simulink model "microgrid_top_fixed_final"  (R2025a)
settings: Solver=ode1  StartTime=0.0  StopTime=T_stop  FixedStep=Ts  RelTol=1e-3
InitFcn:
  | init_microgrid;
values from neighbouring files (symbols this model uses):
  C_dc = 25e-3    (= 0.025)    [init_microgrid.m]
  C_sc = 10    [init_microgrid.m]
  d = par.d    [init_microgrid.m]    (also in make_figures.m = diff([0; on; 0]))
  dt = t(2)-t(1)    [build_chb_inverter.m]    (also in init_microgrid.m = 0.25)
  Emax = 10    [init_microgrid.m]
  eta_inv = 0.96    [init_microgrid.m]
  Ki_ib = Kp_ib*2*pi*fc_i/10    (= 11.8435252813)    [init_microgrid.m]
  Ki_isc = Kp_isc*2*pi*fc_i/10    (= 14.0148382495)    [init_microgrid.m]
  Ki_v = Kp_v*2*pi*fv/10    (= 63.165468167)    [init_microgrid.m]
  Kp_ib = 2*pi*fc_i*L_bat/V_dc_ref    (= 0.00942477796077)    [init_microgrid.m]
  Kp_isc = 2*pi*fc_i*L_sc/V_dc_ref    (= 0.0111526539202)    [init_microgrid.m]
  Kp_v = 2*pi*fv*C_dc*V_dc_ref/V_sc_nom    (= 5.02654824574)    [init_microgrid.m]
  LOAD_SIGN = +1    (= 1)    [init_microgrid.m]
  Pbmax = par.Pb_max    [init_microgrid.m]
  Pmax = max(Ph,[],2)'    [init_microgrid.m]
  prof = Ph'    [init_microgrid.m]    (also in make_figures.m = evalin('base','prof'); end)
  Pscale = 1    [init_microgrid.m]
  Q_sim_Ah = Q_real_Ah*k_scale    (= 0.0180555555556)    [init_microgrid.m]
  R_bat = 0.05    [init_microgrid.m]
  sig = [0.03 0.10 0.15]    [init_microgrid.m]    (also in ppt_plots_pv.m = {Vpv, Ipv, Ppv, Dty, Vbus})
  SoC0 = par.SoC_0    [init_microgrid.m]
  SoC_min = par.SoC_min    [init_microgrid.m]
  T_amb_day = T_amb_cloudy_day; else, G_day = G_clear_day; end    [init_microgrid.m]    (also in run_test1_pv.m = S.T_amb; end\n']))
  t_day = S.t    [init_microgrid.m]
  t_hour = 0.12    [init_microgrid.m]    (also in plot_test4.m = evalin('base','t_hour'); ppt_plots_pv.m = 0.05)
  tau_lpf = 2e-3    (= 0.002)    [init_microgrid.m]
  Tc = 2    [init_microgrid.m]    (also in ppt_plots_pv.m = squeeze(wx.getElement(2).Values.Data))
  th1 = par.th1    [init_microgrid.m]    (also in make_figures.m = 0.05)
  th1_act = th1    [init_microgrid.m]
  th2 = par.th2    [init_microgrid.m]
  th2_act = th2    [init_microgrid.m]
  Ts = Ts_pwr    (= 1e-06)    [init_microgrid.m]
  Ts_ems = t_hour/60    (= 0.002)    [init_microgrid.m]
  Ts_fc = dt*t_hour    (= 0.03)    [init_microgrid.m]
  V_bat_nom = 240    [init_microgrid.m]
  V_dc_ref = 400    [init_microgrid.m]
  V_sc_nom = 250    [init_microgrid.m]
undefined symbols (not defined in the file or in its folder): DiscIntNeverNeededParam, G_day, Ion, Lithium
libraries: spsSeriesRLCBranchLib x9, slpidlib x5, spsVoltageMeasurementLib x5, spsIdealSwitchLib x5, spsIGBTDiodeLib x4, spsCurrentMeasurementLib x3, simulink x3, spsParallelRLCLoadLib x3, spsPWMGeneratorDCDCLib x2, spsDiodeLib x2, spsPVArrayLib x2, spsBatteryLib x1
(part 1 of 2)
settings Model: Creator=mdnih  LastModifiedBy=msssr
settings SolverCC: AutoInsertRateTranBlk=on
settings DebuggingCC: UnconnectedInputMsg=warning

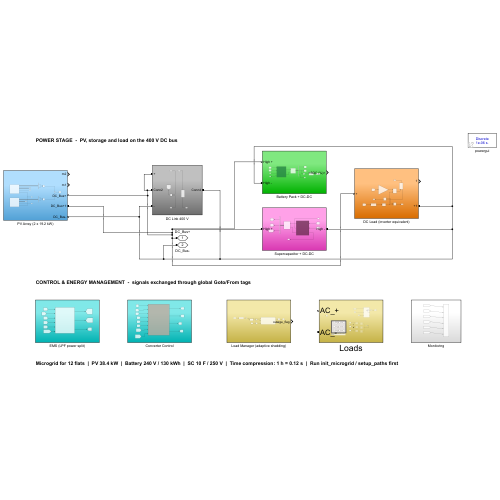
[thumbnail: Simulink's stored preview of the top-level diagram]
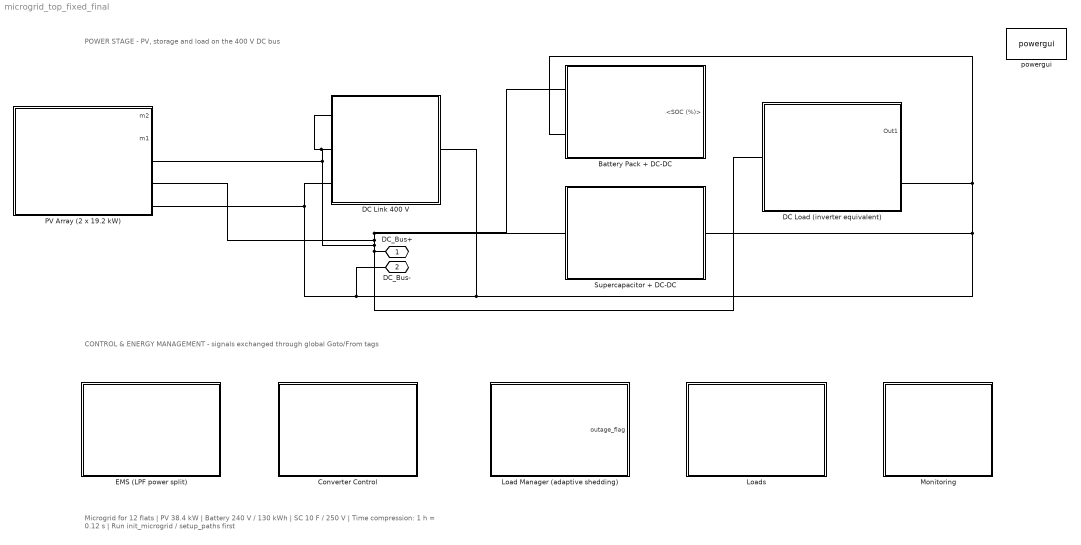
== system microgrid_top_fixed_final ==
  note: POWER STAGE - PV, storage and load on the 400 V DC bus
  note: CONTROL & ENERGY MANAGEMENT - signals exchanged through global Goto/From tags
  note: Microgrid for 12 flats | PV 38.4 kW | Battery 240 V / 130 kWh | SC 10 F / 250 V | Time compression: 1 h = 0.12 s | Run init_microgrid / setup_paths first
  Battery Pack + DC-DC : Subsystem
  Converter Control : Subsystem
  DC Link 400 V : Subsystem
  DC Load (inverter equivalent) : Subsystem
  EMS (LPF power split) : Subsystem
  Load Manager (adaptive shedding) : Subsystem
  Loads : Subsystem
  Monitoring : Subsystem
  PV Array (2 x 19.2 kW) : Subsystem
  Supercapacitor + DC-DC : Subsystem
  powergui : sps_lib/powergui  Priority=1  SimulationMode=Discrete  SampleTime=Ts  frequency=60  Iterations=50  frequencyindice=0  Pbase=100e6  ErrMax=1e-4  UnitsV=kV  UnitsW=MW  buscounter=0  FunctionMessages=off  echomessages=off  EnableUseOfTLC=off  CurrentSourceSwitches=off  DisableSnubberDevices=off  DisableRonSwitches=off  DisableVfSwitches=off  DisplayEquations=off  AutomaticDiscreteSolvers=off  SolverType=Tustin/Backward Euler (TBE)  Interpol=off  ExternalGateDelay=off  methode=off  Ts=100  x0status=blocks  SPID=on  SwTol=0  HookPort=off  NonlinearTolerance=1e-4  nMaxIteration=100  ContinueOnMaxIteration=off  RestoreLinks=warning  ResistiveCurrentMeasurement=off  Frange=[0:2:500]  Ylog=off  Xlog=on  ShowGrid=off  save=off  variable=ZData  structure=0  ZoomFFT=off  StartTime=0.0  cycles=1  DisplayStyle=1  fundamental=60  FreqAxis=off  MaxFrequency=1000  frequencyindicesteady=1  RmsSteady=1  display=off
  DC_Bus+ : PMIOPort  Side=Right
  DC_Bus- : PMIOPort  Port=2  Side=Left
  connections:
  DC Link 400 V/LConn2 -- DC Link 400 V/LConn1 -- PV Array (2 x 19.2 kW)/RConn2 -- Battery Pack + DC-DC/LConn1 -- Supercapacitor + DC-DC/LConn1 -- DC Load (inverter equivalent)/LConn1 -- DC_Bus+/RConn1 -- PV Array (2 x 19.2 kW)/RConn1
  PV Array (2 x 19.2 kW)/RConn3 -- DC Load (inverter equivalent)/RConn1 -- Battery Pack + DC-DC/LConn2 -- Supercapacitor + DC-DC/RConn1 -- DC Link 400 V/RConn1 -- DC_Bus-/RConn1 -- DC Link 400 V/LConn3

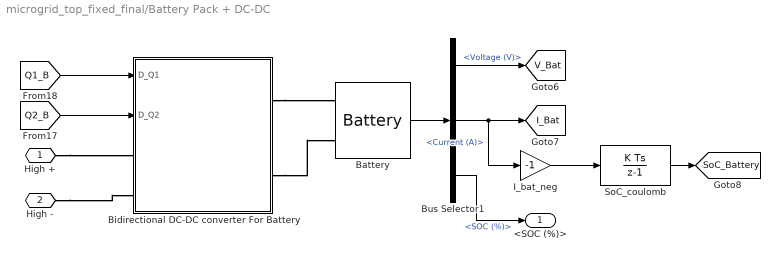
== system microgrid_top_fixed_final/Battery Pack + DC-DC ==
  Battery : spsBatteryLib/Battery  BatType=Lithium-Ion  NomV=V_bat_nom  NomQ=Q_real_Ah  SOC=SoC0*100  Batt_Tr=1e-3  PresetModel=off  MaxQ=Q_real_Ah  MinV=180  FullV=279.3569  Dis_rate=235.5072  R=R_bat  Normal_OP=489.8551  expZone="[259.2926      26.61232]"
      settings: LibrarySourceBlock=electricdrivelib/Extra Sources/Battery
  Bidirectional DC-DC converter For Battery : Subsystem
  Bus Selector1 : BusSelector  OutputSignals=Voltage (V),Current (A),SOC (%)
  I_bat_neg : Gain  Gain=-1
  SoC_coulomb : DiscreteIntegrator  gainval=100/(3600*Q_sim_Ah)  InitialCondition=SoC0*100  SampleTime=Ts  LimitOutput=on  UpperSaturationLimit=100  LowerSaturationLimit=0  ICPrevOutput=DiscIntNeverNeededParam  ICPrevScaledInput=DiscIntNeverNeededParam
  High + : PMIOPort  Side=Left
  High - : PMIOPort  Port=2  Side=Left
  <SOC (%)> : Outport
  tag scope: I_Bat=global, SoC_Battery=global, V_Bat=global
  wires:
  [Q2_B] -> Bidirectional DC-DC converter For Battery/2(D_Q2)
  [Q1_B] -> Bidirectional DC-DC converter For Battery/1(D_Q1)
  Bus Selector1/1 -> [V_Bat]  "<Voltage (V)>"
  I_bat_neg/1 -> SoC_coulomb/1
  Battery/1 -> Bus Selector1/1
  Bus Selector1/2 -> I_bat_neg/1, [I_Bat]  "<Current (A)>"
  Bus Selector1/3 -> <SOC (%)>/1  "<SOC (%)>"
  SoC_coulomb/1 -> [SoC_Battery]
  connections:
  High +/RConn1 -- Bidirectional DC-DC converter For Battery/LConn1
  Bidirectional DC-DC converter For Battery/RConn1 -- Battery/LConn1
  High -/RConn1 -- Bidirectional DC-DC converter For Battery/LConn2
  Bidirectional DC-DC converter For Battery/RConn2 -- Battery/LConn2

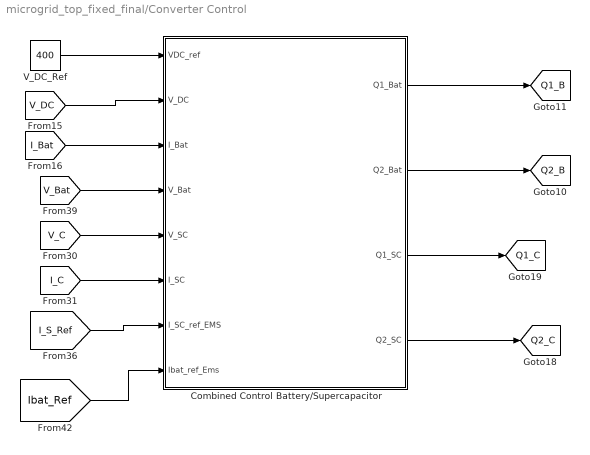
== system microgrid_top_fixed_final/Converter Control ==
  Combined Control Battery/Supercapacitor : Subsystem
  V_DC_Ref : Constant  Value=400
  tag scope: Q1_B=global, Q1_C=global, Q2_B=global, Q2_C=global
  wires:
  [I_C] -> Combined Control Battery/Supercapacitor/6(I_SC)
  [V_DC] -> Combined Control Battery/Supercapacitor/2(V_DC)
  Combined Control Battery/Supercapacitor/4(Q2_SC) -> [Q2_C]
  Combined Control Battery/Supercapacitor/1(Q1_Bat) -> [Q1_B]
  Combined Control Battery/Supercapacitor/3(Q1_SC) -> [Q1_C]
  [I_S_Ref] -> Combined Control Battery/Supercapacitor/7(I_SC_ref_EMS)
  [Ibat_Ref] -> Combined Control Battery/Supercapacitor/8(Ibat_ref_Ems)
  Combined Control Battery/Supercapacitor/2(Q2_Bat) -> [Q2_B]
  V_DC_Ref/1 -> Combined Control Battery/Supercapacitor/1(VDC_ref)
  [I_Bat] -> Combined Control Battery/Supercapacitor/3(I_Bat)
  [V_C] -> Combined Control Battery/Supercapacitor/5("V_SC ")
  [V_Bat] -> Combined Control Battery/Supercapacitor/4(V_Bat)

== system microgrid_top_fixed_final/DC Link 400 V ==
  C_DC_Link : spsSeriesRLCBranchLib/Series RLC Branch  LConnTagsString=__new0  RConnTagsString=__new0  BranchType=C  Resistance=1  Inductance=1e-3  SetiL0=off  InitialCurrent=0  Capacitance=C_dc  Setx0=off  InitialVoltage=0  Measurements=None
  Voltage Measurement : spsVoltageMeasurementLib/Voltage Measurement  PhasorSimulation=off  OutputType=Complex  PSBequivalent=0
  + : PMIOPort  Side=Left
  Conn2 : PMIOPort  Port=2  Side=Left
  - : PMIOPort  Port=3  Side=Left
  Conn4 : PMIOPort  Port=4  Side=Right
  tag scope: V_DC=global
  wires:
  Voltage Measurement/1 -> [V_DC]
  connections:
  C_DC_Link/RConn1 -- Conn4/RConn1
  C_DC_Link/LConn1 -- Conn2/RConn1
  Voltage Measurement/LConn1 -- +/RConn1
  Voltage Measurement/LConn2 -- -/RConn1

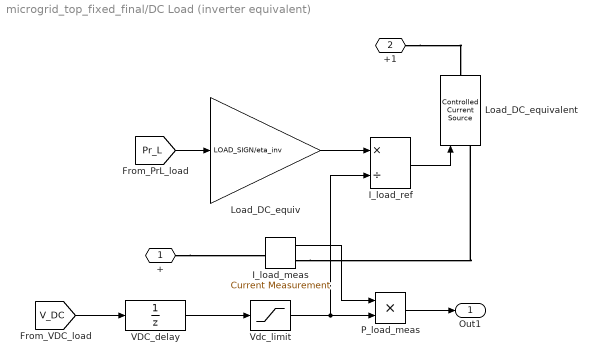
== system microgrid_top_fixed_final/DC Load (inverter equivalent) ==
  I_load_meas : spsCurrentMeasurementLib/Current Measurement  PhasorSimulation=off  OutputType=Complex  PSBequivalent=0
  I_load_ref : Product  Inputs=*/
  Load_DC_equiv : Gain  Gain=LOAD_SIGN/eta_inv
  Load_DC_equivalent : spsControlledCurrentSourceLib/Controlled Current Source  Initialize=on  Source_Type=AC  Amplitude=0  Phase=0  Frequency=0  Measurements=None
  P_load_meas : Product
  VDC_delay : UnitDelay  InitialCondition=V_dc_ref  SampleTime=Ts  HasFrameUpgradeWarning=on
  Vdc_limit : Saturate  UpperLimit=450  LowerLimit=300
  + : PMIOPort  Side=Left
  +1 : PMIOPort  Port=2  Side=Right
  Out1 : Outport
  wires:
  [Pr_L] -> Load_DC_equiv/1
  [V_DC] -> VDC_delay/1
  VDC_delay/1 -> Vdc_limit/1
  Load_DC_equiv/1 -> I_load_ref/1
  I_load_meas/1 -> P_load_meas/1
  Vdc_limit/1 -> I_load_ref/2, P_load_meas/2
  I_load_ref/1 -> Load_DC_equivalent/1
  P_load_meas/1 -> Out1/1
  connections:
  I_load_meas/RConn1 -- Load_DC_equivalent/LConn1
  +/RConn1 -- I_load_meas/LConn1
  +1/RConn1 -- Load_DC_equivalent/RConn1

== system microgrid_top_fixed_final/EMS (LPF power split) ==
  BESS : Subsystem
  tag scope: I_S_Ref=global, Ibat_Ref=global, P_DEF=global
  wires:
  BESS/1(I_BAT_REF) -> [Ibat_Ref]
  [Pr_L] -> BESS/1(P_L)
  [V_Bat] -> BESS/3(V_BAT)
  [P_PV] -> BESS/2(p_pv)
  [I_C] -> BESS/5(I_C)
  [SoC_Battery] -> BESS/6(SOC_Bat)
  [V_C] -> BESS/4(V_C)
  BESS/2(I_S_REF) -> [I_S_Ref]
  BESS/3(P_DEF) -> [P_DEF]

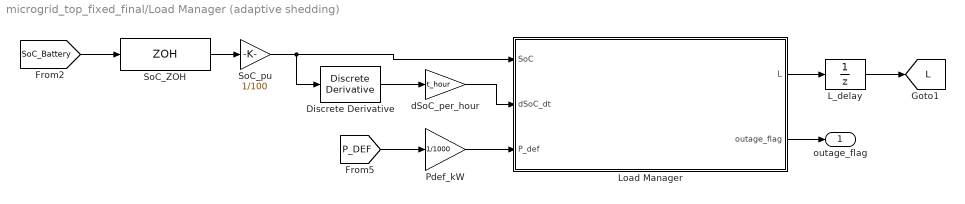
== system microgrid_top_fixed_final/Load Manager (adaptive shedding) ==
  Discrete Derivative : simulink/Discrete/Discrete Derivative  gainval=1.0  ICPrevScaledInput=0.0  OutMin=[]  OutMax=[]  OutDataType=fixdt(1, 16)  OutScaling=2^-10  DoSatur=off
  L_delay : UnitDelay  SampleTime=Ts_ems  HasFrameUpgradeWarning=on
  Load Manager : Stateflow chart  TreatAsAtomicUnit=on
  Pdef_kW : Gain  Gain=1/1000
  SoC_ZOH : ZeroOrderHold  SampleTime=Ts_ems
  SoC_pu : Gain  Gain=1/100
  dSoC_per_hour : Gain  Gain=t_hour
  outage_flag : Outport
  tag scope: L=global
  wires:
  Discrete Derivative/1 -> dSoC_per_hour/1
  [SoC_Battery] -> SoC_ZOH/1
  SoC_ZOH/1 -> SoC_pu/1
  Pdef_kW/1 -> Load Manager/3(P_def)
  SoC_pu/1 -> Load Manager/1(SoC), Discrete Derivative/1
  [P_DEF] -> Pdef_kW/1
  dSoC_per_hour/1 -> Load Manager/2(dSoC_dt)
  Load Manager/1(L) -> L_delay/1
  Load Manager/2(outage_flag) -> outage_flag/1
  L_delay/1 -> [L]

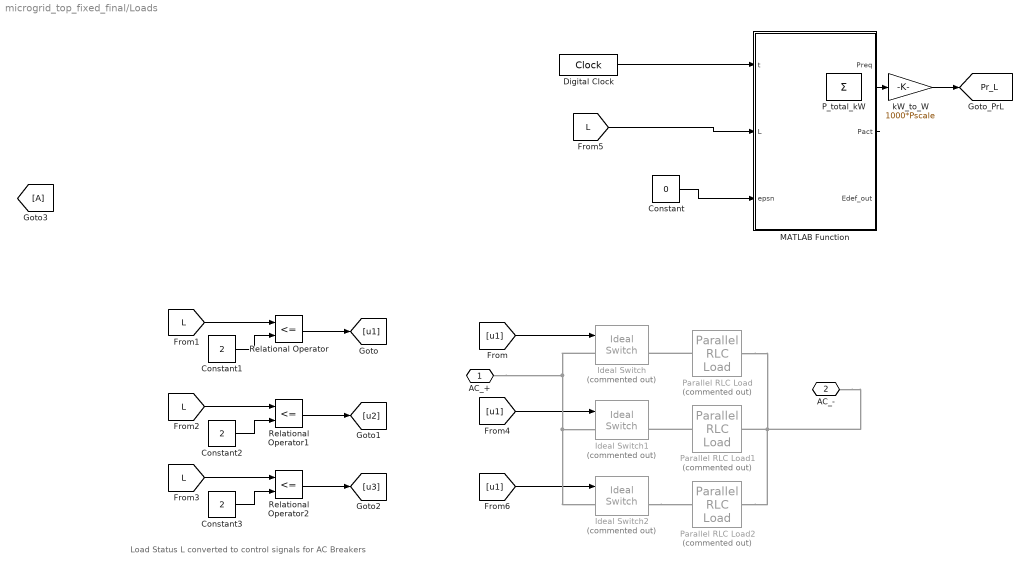
== system microgrid_top_fixed_final/Loads ==
  note: Load Status L converted to control signals
      | for AC Breakers
  Constant : Constant  Value=0
  Constant1 : Constant  Value=2
  Constant2 : Constant  Value=2
  Constant3 : Constant  Value=2
  Digital Clock : DigitalClock  SampleTime=Ts_fc
  Goto3 : Goto
  Ideal Switch : spsIdealSwitchLib/Ideal Switch  Commented=on  Ron=0.001  Lon=0  IC=0  Rs=1e5  Cs=inf  Measurements=on
  Ideal Switch1 : spsIdealSwitchLib/Ideal Switch  Commented=on  Ron=0.001  Lon=0  IC=0  Rs=1e5  Cs=inf  Measurements=on
  Ideal Switch2 : spsIdealSwitchLib/Ideal Switch  Commented=on  Ron=0.001  Lon=0  IC=0  Rs=1e5  Cs=inf  Measurements=on
  MATLAB Function : MATLAB Function  TreatAsAtomicUnit=on
  P_total_kW : Sum  Inputs=+
  Parallel RLC Load : spsParallelRLCLoadLib/Parallel RLC Load  Commented=on  LConnTagsString=a  RConnTagsString=__new0  NominalVoltage=1000  NominalFrequency=60  ActivePower=10e3  InductivePower=100  CapacitivePower=100  Setx0=off  InitialVoltage=0  SetiL0=off  InitialCurrent=0  Measurements=None  LoadType=constant Z
      settings: AttributesFormatString=\n  LibrarySourceBlock=sps_lib/Passives/Parallel RLC Load
  Parallel RLC Load1 : spsParallelRLCLoadLib/Parallel RLC Load  Commented=on  LConnTagsString=a  RConnTagsString=__new0  NominalVoltage=1000  NominalFrequency=60  ActivePower=10e3  InductivePower=100  CapacitivePower=100  Setx0=off  InitialVoltage=0  SetiL0=off  InitialCurrent=0  Measurements=None  LoadType=constant Z
      settings: AttributesFormatString=\n  LibrarySourceBlock=sps_lib/Passives/Parallel RLC Load
  Parallel RLC Load2 : spsParallelRLCLoadLib/Parallel RLC Load  Commented=on  LConnTagsString=a  RConnTagsString=__new0  NominalVoltage=1000  NominalFrequency=60  ActivePower=10e3  InductivePower=100  CapacitivePower=100  Setx0=off  InitialVoltage=0  SetiL0=off  InitialCurrent=0  Measurements=None  LoadType=constant Z
      settings: AttributesFormatString=\n  LibrarySourceBlock=sps_lib/Passives/Parallel RLC Load
  Relational Operator : RelationalOperator  Operator=<=  OutDataTypeStr=boolean  RndMeth=Simplest  InputSameDT=off
  Relational Operator1 : RelationalOperator  Operator=<=  OutDataTypeStr=boolean  RndMeth=Simplest  InputSameDT=off
  Relational Operator2 : RelationalOperator  Operator=<=  OutDataTypeStr=boolean  RndMeth=Simplest  InputSameDT=off
  kW_to_W : Gain  Gain=1000*Pscale
  AC_+ : PMIOPort  Side=Left
  AC_- : PMIOPort  Port=2  Side=Left
  tag scope: Pr_L=global
  wires:
  Digital Clock/1 -> MATLAB Function/1(t)
  [L] -> MATLAB Function/2(L)
  Constant/1 -> MATLAB Function/3(epsn)
  [L] -> Relational Operator/1
  Constant1/1 -> Relational Operator/2
  Constant2/1 -> Relational Operator1/2
  [L] -> Relational Operator1/1
  [L] -> Relational Operator2/1
  Constant3/1 -> Relational Operator2/2
  Relational Operator/1 -> [u1]
  Relational Operator2/1 -> [u3]
  Relational Operator1/1 -> [u2]
  [u1] -> Ideal Switch/1
  [u1] -> Ideal Switch1/1
  [u1] -> Ideal Switch2/1
  MATLAB Function/2(Pact) -> P_total_kW/1
  P_total_kW/1 -> kW_to_W/1
  kW_to_W/1 -> [Pr_L]
  connections:
  Ideal Switch/LConn1 -- Ideal Switch2/LConn1 -- Ideal Switch1/LConn1 -- AC_+/RConn1
  Parallel RLC Load/LConn1 -- Ideal Switch/RConn1
  Parallel RLC Load1/LConn1 -- Ideal Switch1/RConn1
  Ideal Switch2/RConn1 -- Parallel RLC Load2/LConn1
  Parallel RLC Load/RConn1 -- AC_-/RConn1 -- Parallel RLC Load1/RConn1 -- Parallel RLC Load2/RConn1

== system microgrid_top_fixed_final/Monitoring ==
  System Scope : Scope  NumInputPorts=6
      settings: ActiveDisplayYMinimum=89.7017199795797  ActiveDisplayYMaximum=442.12734403903488
  wires:
  [V_DC] -> System Scope/1
  [V_Bat] -> System Scope/2
  [SoC_Battery] -> System Scope/3
  [P_PV] -> System Scope/4
  [Pr_L] -> System Scope/5
  [L] -> System Scope/6

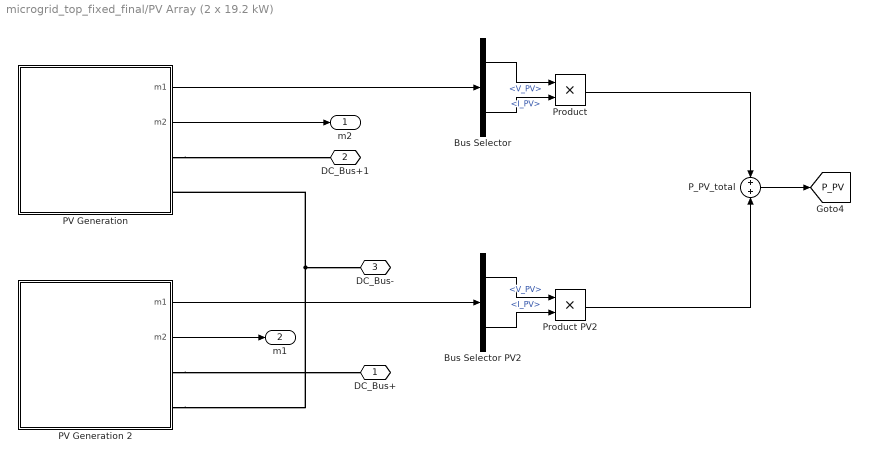
== system microgrid_top_fixed_final/PV Array (2 x 19.2 kW) ==
  Bus Selector : BusSelector  OutputSignals=V_PV,I_PV
  Bus Selector PV2 : BusSelector  OutputSignals=V_PV,I_PV
  PV Generation : Subsystem
  PV Generation 2 : Subsystem
  P_PV_total : Sum
  Product : Product
  Product PV2 : Product
  DC_Bus+ : PMIOPort  Side=Right
  DC_Bus+1 : PMIOPort  Port=2  Side=Right
  DC_Bus- : PMIOPort  Port=3  Side=Right
  m2 : Outport
  m1 : Outport  Port=2
  tag scope: P_PV=global
  wires:
  P_PV_total/1 -> [P_PV]
  Bus Selector PV2/2 -> Product PV2/2  "<I_PV>"
  PV Generation 2/1(m1) -> Bus Selector PV2/1
  PV Generation 2/2(m2) -> m1/1
  PV Generation/2(m2) -> m2/1
  PV Generation/1(m1) -> Bus Selector/1
  Bus Selector PV2/1 -> Product PV2/1  "<V_PV>"
  Product PV2/1 -> P_PV_total/2
  Bus Selector/1 -> Product/1  "<V_PV>"
  Bus Selector/2 -> Product/2  "<I_PV>"
  Product/1 -> P_PV_total/1
  connections:
  PV Generation 2/RConn1 -- DC_Bus+/RConn1
  PV Generation 2/RConn2 -- PV Generation/RConn2 -- DC_Bus-/RConn1
  PV Generation/RConn1 -- DC_Bus+1/RConn1

== system microgrid_top_fixed_final/Supercapacitor + DC-DC ==
  Bidirectional DC-DC converter For Supercapacitor : Subsystem
  Bus Selector2 : BusSelector  OutputSignals=Voltage V,Current I,SOC %
  Supercapacitor : spsSupercapacitorLib/Supercapacitor  C=C_sc  Rdc=0.003  Voltage=V_sc_nom  Ns=1  Np=1  Vinit=V_sc_init  Temp=25  Nc=1  r=1e-9  epsilon=6.0208e-10  Ioc=10  Vself="[48  47.8  47.06  44.65]"
      settings: LibrarySourceBlock=electricdrivelib/Extra Sources/Supercapacitor
  High + : PMIOPort  Side=Left
  High - : PMIOPort  Port=2  Side=Right
  tag scope: I_C=global, SoC_Cap=global, V_C=global
  wires:
  Bus Selector2/3 -> [SoC_Cap]  "<SOC %>"
  Bus Selector2/2 -> [I_C]  "<Current I>"
  Supercapacitor/1 -> Bus Selector2/1
  Bus Selector2/1 -> [V_C]  "<Voltage V>"
  [Q1_C] -> Bidirectional DC-DC converter For Supercapacitor/1(D_Q1)
  [Q2_C] -> Bidirectional DC-DC converter For Supercapacitor/2(D_Q2)
  connections:
  High -/RConn1 -- Bidirectional DC-DC converter For Supercapacitor/RConn2
  High +/RConn1 -- Bidirectional DC-DC converter For Supercapacitor/LConn1
  Supercapacitor/LConn1 -- Bidirectional DC-DC converter For Supercapacitor/RConn1
  Supercapacitor/LConn2 -- Bidirectional DC-DC converter For Supercapacitor/RConn3

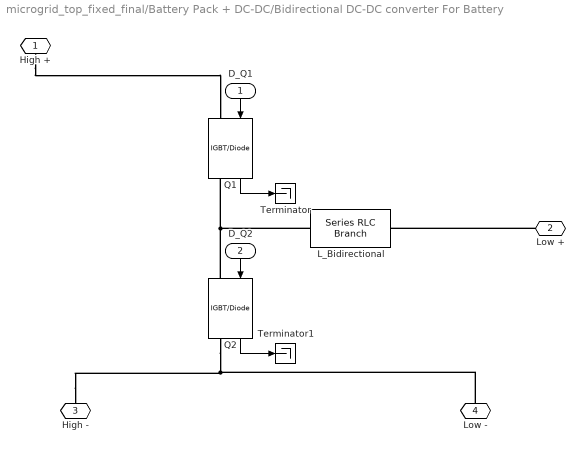
== system microgrid_top_fixed_final/Battery Pack + DC-DC/Bidirectional DC-DC converter For Battery ==
  D_Q1 : Inport
  D_Q2 : Inport  Port=2
  L_Bidirectional : spsSeriesRLCBranchLib/Series RLC Branch  LConnTagsString=__new0  RConnTagsString=__new0  BranchType=RL  Resistance=0.05  Inductance=0.3e-3  SetiL0=off  InitialCurrent=0  Capacitance=1e-6  Setx0=off  InitialVoltage=0  Measurements=None
  Q1 : spsIGBTDiodeLib/IGBT//Diode  Ron=1e-3  Rs=1e5  Cs=inf  Measurements=on
  Q2 : spsIGBTDiodeLib/IGBT//Diode  Ron=1e-3  Rs=1e5  Cs=inf  Measurements=on
  Terminator : Terminator
  Terminator1 : Terminator
  High + : PMIOPort  Side=Left
  Low + : PMIOPort  Port=2  Side=Right
  High - : PMIOPort  Port=3  Side=Left
  Low - : PMIOPort  Port=4  Side=Right
  wires:
  D_Q2/1 -> Q2/1
  D_Q1/1 -> Q1/1
  Q1/1 -> Terminator/1
  Q2/1 -> Terminator1/1
  connections:
  High -/RConn1 -- Low -/RConn1 -- Q2/RConn1
  High +/RConn1 -- Q1/LConn1
  Low +/RConn1 -- L_Bidirectional/RConn1
  Q2/LConn1 -- L_Bidirectional/LConn1 -- Q1/RConn1

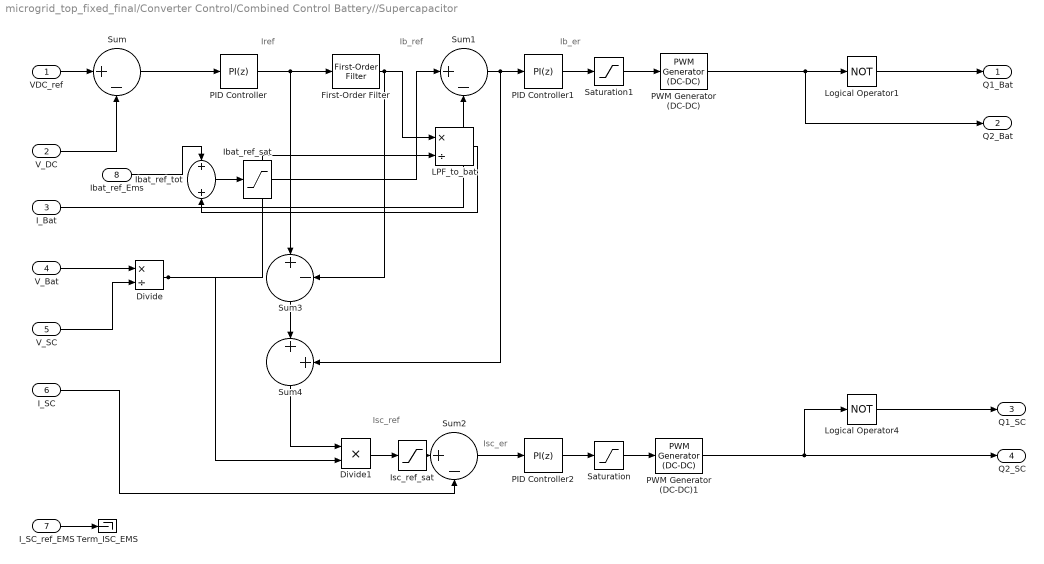
== system microgrid_top_fixed_final/Converter Control/Combined Control Battery//Supercapacitor ==
  note: Isc_er
  note: Isc_ref
  note: Ib_er
  note: Ib_ref
  note: Iref
  VDC_ref : Inport
  V_DC : Inport  Port=2
  I_Bat : Inport  Port=3
  V_Bat : Inport  Port=4
  "V_SC " : Inport  Port=5
  I_SC : Inport  Port=6
  I_SC_ref_EMS : Inport  Port=7
  Ibat_ref_Ems : Inport  Port=8
  Divide : Product  Inputs=*/
  Divide1 : Product  Inputs=**
  First-Order Filter : spsFirstOrderFilterLib/First-Order Filter  FilterType=Lowpass  Tc=0.015  Ts=Ts  Initialize=off  Vac_Init=[0, 0, 60]  Vdc_Init=0  PlotResponse=off  FreqRange="[0,  200,  1]"
  Ibat_ref_sat : Saturate  UpperLimit=1.5*Pbmax*1e3/V_bat_nom  LowerLimit=-(1.5*Pbmax*1e3/V_bat_nom)
  Ibat_ref_tot : Sum
  Isc_ref_sat : Saturate  UpperLimit=200  LowerLimit=-(200)
  LPF_to_bat : Product  Inputs=*/
  Logical Operator1 : Logic  Operator=NOT  AllPortsSameDT=off  OutDataTypeStr=boolean
  Logical Operator4 : Logic  Operator=NOT  AllPortsSameDT=off  OutDataTypeStr=boolean
  PID Controller : slpidlib/PID Controller  Controller=PI  Form=Parallel  TimeDomain=Discrete-time  UseExternalTs=off  SampleTime=Ts  IntegratorMethod=Backward Euler  FilterMethod=Backward Euler  ControllerParametersSource=internal  P=Kp_v  I=Ki_v  UseKiTs=off  D=0  UseExternalDerivativeSource=off  N=100  UseFilter=on  TunerSelectOption=Transfer Function Based (PID Tuner App)  InitialConditionSource=internal  InitialConditionForIntegrator=0  InitialConditionForFilter=0  DifferentiatorICPrevScaledInput=0  ExternalReset=none  TrackingMode=off  Kt=1  LimitOutput=on  SatLimitsSource=internal  UpperSaturationLimit=1.5*Pbmax*1e3/V_bat_nom + 200  LowerSaturationLimit=-(1.5*Pbmax*1e3/V_bat_nom + 200)  LinearizeAsGain=on  AntiWindupMode=clamping  Kb=1  LimitIntegrator=off  UpperIntegratorSaturationLimit=inf  LowerIntegratorSaturationLimit=-inf  POutMin=[]  POutMax=[]  IOutMin=[]  IOutMax=[]  DOutMin=[]  DOutMax=[]  NOutMin=[]  NOutMax=[]  SumOutMin=[]  SumOutMax=[]  SaturationOutMin=[]  SaturationOutMax=[]  PParamMin=[]  PParamMax=[]  IParamMin=[]  IParamMax=[]  DParamMin=[]  DParamMax=[]  NParamMin=[]  NParamMax=[]  KbParamMin=[]  KbParamMax=[]  KtParamMin=[]  KtParamMax=[]  KbOutMin=[]  KbOutMax=[]  KtOutMin=[]  KtOutMax=[]  IntegratorOutMin=[]  IntegratorOutMax=[]  FilterOutMin=[]  FilterOutMax=[]  SumI1OutMin=[]  SumI1OutMax=[]  SumI2OutMin=[]  SumI2OutMax=[]  SumI3OutMin=[]  SumI3OutMax=[]  SumI4OutMin=[]  SumI4OutMax=[]  SumDOutMin=[]  SumDOutMax=[]  DifferentiatorOutMin=[]  DifferentiatorOutMax=[]  FilterDiffOutCoefMin=[]  FilterDiffOutCoefMax=[]  ReciprocalOutMin=[]  ReciprocalOutMax=[]  SumDenOutMin=[]  SumDenOutMax=[]  SumNumOutMin=[]  SumNumOutMax=[]  DivideOutMin=[]  DivideOutMax=[]  UdiffTsProdOutMin=[]  UdiffTsProdOutMax=[]  NTsProdOutMin=[]  NTsProdOutMax=[]  UintegralTsProdOutMin=[]  UintegralTsProdOutMax=[]  UngainTsProdOutMin=[]  UngainTsProdOutMax=[]  ClampingZeroOutDataTypeStr=Inherit: Inherit via back propagation  ClampingZeroOutMin=[]  ClampingZeroOutMax=[]  FilterDenConstantOutDataTypeStr=Inherit: Inherit via back propagation  FilterDenConstantOutMin=[]  FilterDenConstantOutMax=[]  PCopyOutDataTypeStr=Inherit: Inherit via back propagation  PCopyOutMin=[]  PCopyOutMax=[]  NCopyOutDataTypeStr=Inherit: Inherit via back propagation  NCopyOutMin=[]  NCopyOutMax=[]  IntegratorContinuousStateAttributes=''  IntegratorStateMustResolveToSignalObject=off  IntegratorRTWStateStorageClass=Auto  FilterContinuousStateAttributes=''  FilterStateMustResolveToSignalObject=off  FilterRTWStateStorageClass=Auto  ParallelPVariant=InternalParameters  IdealPVariant=Disabled  IVariant=InternalParameters  DVariant=Disabled  IntegratorVariant=Discrete  SatVariant=Enabled  AWVariant=DiscClampingParallel  PCopyVariant=Disabled  TRVariant=Disabled  FdbkBlocksVariant=Feedback  IdealPFdbkVariant=Passthrough  SatFdbkVariant=Passthrough  DerivativeFilterVariant=Disabled  NVariant=Disabled  NCopyVariant=Disabled_SignalSpec  FilterICVariant=Disabled  IntegratorICVariant=InternalICs  ExternalResetVariant=Disabled  TRSumVariant=Passthrough  SumFdbkVariant=Enabled  SumVariant=Sum_PI  TsampFilterVariant=InternalTs  TsampNgainVariant=Passthrough  TsampIntegralVariant=Disabled_SignalSpec  ExternalSaturationOutDataTypeStr=Inherit: Same as second input  DerivativeSourceVariant=Disabled  PreIntVariant=InternalPreInt
  PID Controller1 : slpidlib/PID Controller  Controller=PI  Form=Parallel  TimeDomain=Discrete-time  UseExternalTs=off  SampleTime=Ts  IntegratorMethod=Backward Euler  FilterMethod=Backward Euler  ControllerParametersSource=internal  P=Kp_ib  I=Ki_ib  UseKiTs=off  D=0  UseExternalDerivativeSource=off  N=100  UseFilter=on  TunerSelectOption=Transfer Function Based (PID Tuner App)  InitialConditionSource=internal  InitialConditionForIntegrator=0  InitialConditionForFilter=0  DifferentiatorICPrevScaledInput=0  ExternalReset=none  TrackingMode=off  Kt=1  LimitOutput=on  SatLimitsSource=internal  UpperSaturationLimit=0.9  LowerSaturationLimit=0  LinearizeAsGain=on  AntiWindupMode=clamping  Kb=1  LimitIntegrator=off  UpperIntegratorSaturationLimit=inf  LowerIntegratorSaturationLimit=-inf  POutMin=[]  POutMax=[]  IOutMin=[]  IOutMax=[]  DOutMin=[]  DOutMax=[]  NOutMin=[]  NOutMax=[]  SumOutMin=[]  SumOutMax=[]  SaturationOutMin=[]  SaturationOutMax=[]  PParamMin=[]  PParamMax=[]  IParamMin=[]  IParamMax=[]  DParamMin=[]  DParamMax=[]  NParamMin=[]  NParamMax=[]  KbParamMin=[]  KbParamMax=[]  KtParamMin=[]  KtParamMax=[]  KbOutMin=[]  KbOutMax=[]  KtOutMin=[]  KtOutMax=[]  IntegratorOutMin=[]  IntegratorOutMax=[]  FilterOutMin=[]  FilterOutMax=[]  SumI1OutMin=[]  SumI1OutMax=[]  SumI2OutMin=[]  SumI2OutMax=[]  SumI3OutMin=[]  SumI3OutMax=[]  SumI4OutMin=[]  SumI4OutMax=[]  SumDOutMin=[]  SumDOutMax=[]  DifferentiatorOutMin=[]  DifferentiatorOutMax=[]  FilterDiffOutCoefMin=[]  FilterDiffOutCoefMax=[]  ReciprocalOutMin=[]  ReciprocalOutMax=[]  SumDenOutMin=[]  SumDenOutMax=[]  SumNumOutMin=[]  SumNumOutMax=[]  DivideOutMin=[]  DivideOutMax=[]  UdiffTsProdOutMin=[]  UdiffTsProdOutMax=[]  NTsProdOutMin=[]  NTsProdOutMax=[]  UintegralTsProdOutMin=[]  UintegralTsProdOutMax=[]  UngainTsProdOutMin=[]  UngainTsProdOutMax=[]  ClampingZeroOutDataTypeStr=Inherit: Inherit via back propagation  ClampingZeroOutMin=[]  ClampingZeroOutMax=[]  FilterDenConstantOutDataTypeStr=Inherit: Inherit via back propagation  FilterDenConstantOutMin=[]  FilterDenConstantOutMax=[]  PCopyOutDataTypeStr=Inherit: Inherit via back propagation  PCopyOutMin=[]  PCopyOutMax=[]  NCopyOutDataTypeStr=Inherit: Inherit via back propagation  NCopyOutMin=[]  NCopyOutMax=[]  IntegratorContinuousStateAttributes=''  IntegratorStateMustResolveToSignalObject=off  IntegratorRTWStateStorageClass=Auto  FilterContinuousStateAttributes=''  FilterStateMustResolveToSignalObject=off  FilterRTWStateStorageClass=Auto  ParallelPVariant=InternalParameters  IdealPVariant=Disabled  IVariant=InternalParameters  DVariant=Disabled  IntegratorVariant=Discrete  SatVariant=Enabled  AWVariant=DiscClampingParallel  PCopyVariant=Disabled  TRVariant=Disabled  FdbkBlocksVariant=Feedback  IdealPFdbkVariant=Passthrough  SatFdbkVariant=Passthrough  DerivativeFilterVariant=Disabled  NVariant=Disabled  NCopyVariant=Disabled_SignalSpec  FilterICVariant=Disabled  IntegratorICVariant=InternalICs  ExternalResetVariant=Disabled  TRSumVariant=Passthrough  SumFdbkVariant=Enabled  SumVariant=Sum_PI  TsampFilterVariant=InternalTs  TsampNgainVariant=Passthrough  TsampIntegralVariant=Disabled_SignalSpec  ExternalSaturationOutDataTypeStr=Inherit: Same as second input  DerivativeSourceVariant=Disabled  PreIntVariant=InternalPreInt
  PID Controller2 : slpidlib/PID Controller  Controller=PI  Form=Parallel  TimeDomain=Discrete-time  UseExternalTs=off  SampleTime=Ts  IntegratorMethod=Backward Euler  FilterMethod=Backward Euler  ControllerParametersSource=internal  P=Kp_isc  I=Ki_isc  UseKiTs=off  D=0  UseExternalDerivativeSource=off  N=100  UseFilter=on  TunerSelectOption=Transfer Function Based (PID Tuner App)  InitialConditionSource=internal  InitialConditionForIntegrator=0  InitialConditionForFilter=0  DifferentiatorICPrevScaledInput=0  ExternalReset=none  TrackingMode=off  Kt=1  LimitOutput=on  SatLimitsSource=internal  UpperSaturationLimit=0.9  LowerSaturationLimit=0  LinearizeAsGain=on  AntiWindupMode=clamping  Kb=1  LimitIntegrator=off  UpperIntegratorSaturationLimit=inf  LowerIntegratorSaturationLimit=-inf  POutMin=[]  POutMax=[]  IOutMin=[]  IOutMax=[]  DOutMin=[]  DOutMax=[]  NOutMin=[]  NOutMax=[]  SumOutMin=[]  SumOutMax=[]  SaturationOutMin=[]  SaturationOutMax=[]  PParamMin=[]  PParamMax=[]  IParamMin=[]  IParamMax=[]  DParamMin=[]  DParamMax=[]  NParamMin=[]  NParamMax=[]  KbParamMin=[]  KbParamMax=[]  KtParamMin=[]  KtParamMax=[]  KbOutMin=[]  KbOutMax=[]  KtOutMin=[]  KtOutMax=[]  IntegratorOutMin=[]  IntegratorOutMax=[]  FilterOutMin=[]  FilterOutMax=[]  SumI1OutMin=[]  SumI1OutMax=[]  SumI2OutMin=[]  SumI2OutMax=[]  SumI3OutMin=[]  SumI3OutMax=[]  SumI4OutMin=[]  SumI4OutMax=[]  SumDOutMin=[]  SumDOutMax=[]  DifferentiatorOutMin=[]  DifferentiatorOutMax=[]  FilterDiffOutCoefMin=[]  FilterDiffOutCoefMax=[]  ReciprocalOutMin=[]  ReciprocalOutMax=[]  SumDenOutMin=[]  SumDenOutMax=[]  SumNumOutMin=[]  SumNumOutMax=[]  DivideOutMin=[]  DivideOutMax=[]  UdiffTsProdOutMin=[]  UdiffTsProdOutMax=[]  NTsProdOutMin=[]  NTsProdOutMax=[]  UintegralTsProdOutMin=[]  UintegralTsProdOutMax=[]  UngainTsProdOutMin=[]  UngainTsProdOutMax=[]  ClampingZeroOutDataTypeStr=Inherit: Inherit via back propagation  ClampingZeroOutMin=[]  ClampingZeroOutMax=[]  FilterDenConstantOutDataTypeStr=Inherit: Inherit via back propagation  FilterDenConstantOutMin=[]  FilterDenConstantOutMax=[]  PCopyOutDataTypeStr=Inherit: Inherit via back propagation  PCopyOutMin=[]  PCopyOutMax=[]  NCopyOutDataTypeStr=Inherit: Inherit via back propagation  NCopyOutMin=[]  NCopyOutMax=[]  IntegratorContinuousStateAttributes=''  IntegratorStateMustResolveToSignalObject=off  IntegratorRTWStateStorageClass=Auto  FilterContinuousStateAttributes=''  FilterStateMustResolveToSignalObject=off  FilterRTWStateStorageClass=Auto  ParallelPVariant=InternalParameters  IdealPVariant=Disabled  IVariant=InternalParameters  DVariant=Disabled  IntegratorVariant=Discrete  SatVariant=Enabled  AWVariant=DiscClampingParallel  PCopyVariant=Disabled  TRVariant=Disabled  FdbkBlocksVariant=Feedback  IdealPFdbkVariant=Passthrough  SatFdbkVariant=Passthrough  DerivativeFilterVariant=Disabled  NVariant=Disabled  NCopyVariant=Disabled_SignalSpec  FilterICVariant=Disabled  IntegratorICVariant=InternalICs  ExternalResetVariant=Disabled  TRSumVariant=Passthrough  SumFdbkVariant=Enabled  SumVariant=Sum_PI  TsampFilterVariant=InternalTs  TsampNgainVariant=Passthrough  TsampIntegralVariant=Disabled_SignalSpec  ExternalSaturationOutDataTypeStr=Inherit: Same as second input  DerivativeSourceVariant=Disabled  PreIntVariant=InternalPreInt
  PWM Generator (DC-DC) : spsPWMGeneratorDCDCLib/PWM Generator (DC-DC)  Fsw=f_sw  Ts=Ts
  PWM Generator (DC-DC)1 : spsPWMGeneratorDCDCLib/PWM Generator (DC-DC)  Fsw=f_sw  Ts=Ts
  Saturation : Saturate  UpperLimit=0.9  LowerLimit=0
  Saturation1 : Saturate  UpperLimit=0.9  LowerLimit=0
  Sum{,1..3} (4 alike) : Sum  Inputs=|+-
  Sum4 : Sum  Inputs=|++
  Term_ISC_EMS : Terminator
  Q1_Bat : Outport
  Q2_Bat : Outport  Port=2
  Q1_SC : Outport  Port=3
  Q2_SC : Outport  Port=4
  wires:
  Sum1/1 -> PID Controller1/1, Sum4/2
  PWM Generator (DC-DC)/1 -> Logical Operator1/1, Q2_Bat/1
  I_Bat/1 -> Sum1/2
  I_SC/1 -> Sum2/2
  Sum2/1 -> PID Controller2/1
  Logical Operator1/1 -> Q1_Bat/1
  Sum/1 -> PID Controller/1
  VDC_ref/1 -> Sum/1
  V_DC/1 -> Sum/2
  V_Bat/1 -> Divide/1
  "V_SC "/1 -> Divide/2
  Logical Operator4/1 -> Q1_SC/1
  PWM Generator (DC-DC)1/1 -> Q2_SC/1, Logical Operator4/1
  PID Controller/1 -> First-Order Filter/1, Sum3/1
  Sum3/1 -> Sum4/1
  Divide/1 -> Divide1/2, LPF_to_bat/2
  Sum4/1 -> Divide1/1
  PID Controller2/1 -> Saturation/1
  Saturation/1 -> PWM Generator (DC-DC)1/1
  PID Controller1/1 -> Saturation1/1
  Saturation1/1 -> PWM Generator (DC-DC)/1
  First-Order Filter/1 -> Sum3/2, LPF_to_bat/1
  I_SC_ref_EMS/1 -> Term_ISC_EMS/1
  Ibat_ref_Ems/1 -> Ibat_ref_tot/1
  LPF_to_bat/1 -> Ibat_ref_tot/2
  Ibat_ref_tot/1 -> Ibat_ref_sat/1
  Ibat_ref_sat/1 -> Sum1/1
  Divide1/1 -> Isc_ref_sat/1
  Isc_ref_sat/1 -> Sum2/1

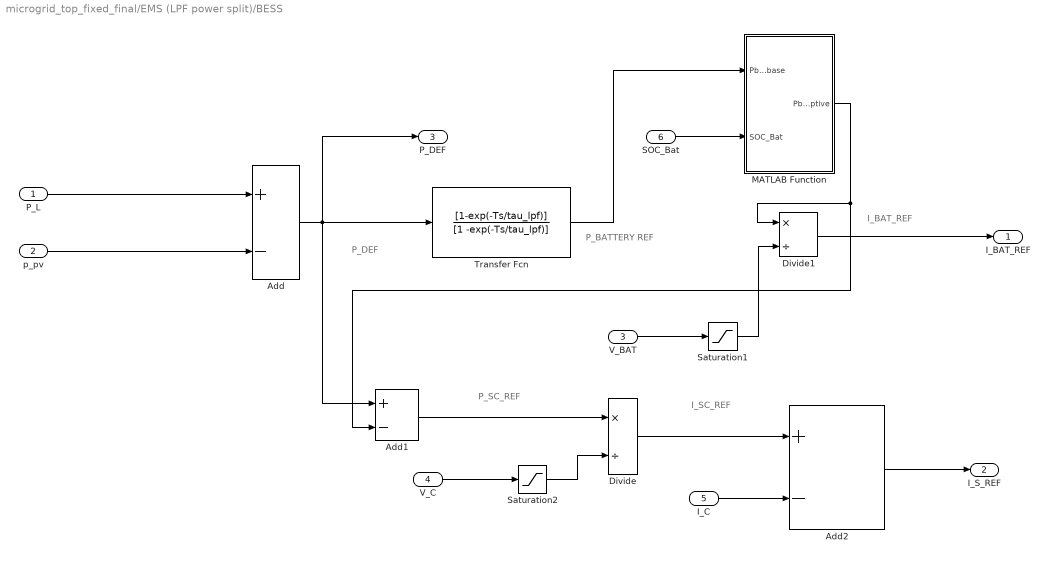
== system microgrid_top_fixed_final/EMS (LPF power split)/BESS ==
  note: P_SC_REF
  note: I_BAT_REF
  note: P_DEF
  note: P_BATTERY REF
  note: I_SC_REF
  P_L : Inport
  p_pv : Inport  Port=2
  V_BAT : Inport  Port=3
  V_C : Inport  Port=4
  I_C : Inport  Port=5
  SOC_Bat : Inport  Port=6
  Add : Sum  Inputs=+-
  Add1 : Sum  Inputs=+-
  Add2 : Sum  Inputs=+-
  Divide : Product  Inputs=*/
  Divide1 : Product  Inputs=*/
  MATLAB Function : MATLAB Function  TreatAsAtomicUnit=on
  Saturation1 : Saturate  UpperLimit=1000  LowerLimit=1
  Saturation2 : Saturate  UpperLimit=1000  LowerLimit=1
  Transfer Fcn : DiscreteTransferFcn  Numerator=[1-exp(-Ts/tau_lpf)]  Denominator=[1 -exp(-Ts/tau_lpf)]  SampleTime=Ts
  I_BAT_REF : Outport
  I_S_REF : Outport  Port=2
  P_DEF : Outport  Port=3
  wires:
  Transfer Fcn/1 -> MATLAB Function/1(Pbat_base)
  Add1/1 -> Divide/1
  Saturation2/1 -> Divide/2
  MATLAB Function/1(Pbat_adaptive) -> Add1/2, Divide1/1
  Add/1 -> P_DEF/1, Transfer Fcn/1, Add1/1
  Saturation1/1 -> Divide1/2
  Divide/1 -> Add2/1
  P_L/1 -> Add/1
  p_pv/1 -> Add/2
  SOC_Bat/1 -> MATLAB Function/2(SOC_Bat)
  Divide1/1 -> I_BAT_REF/1
  Add2/1 -> I_S_REF/1
  V_BAT/1 -> Saturation1/1
  I_C/1 -> Add2/2
  V_C/1 -> Saturation2/1

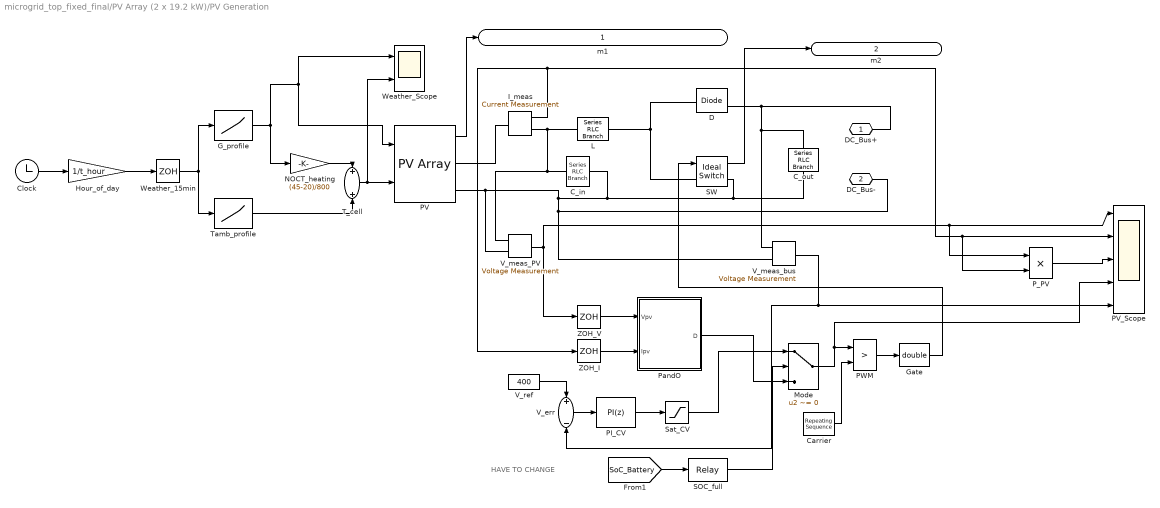
== system microgrid_top_fixed_final/PV Array (2 x 19.2 kW)/PV Generation ==
  note: HAVE TO CHANGE
  C_in : spsSeriesRLCBranchLib/Series RLC Branch  LConnTagsString=__new0  RConnTagsString=__new0  BranchType=C  Resistance=1  Inductance=1e-3  SetiL0=off  InitialCurrent=0  Capacitance=270e-6  Setx0=off  InitialVoltage=0  Measurements=None
  C_out : spsSeriesRLCBranchLib/Series RLC Branch  LConnTagsString=__new0  RConnTagsString=__new0  BranchType=C  Resistance=1  Inductance=1e-3  SetiL0=off  InitialCurrent=0  Capacitance=270e-6  Setx0=off  InitialVoltage=0  Measurements=None
  Carrier : simulink/Sources/Repeating Sequence  rep_seq_t=[0 5e-05]  rep_seq_y=[0 1]
  Clock : Clock
  D : spsDiodeLib/Diode  Ron=0.001  Lon=0  Vf=0.8  IC=0  UseSnubber=0  Rs=500  Cs=250e-9  Measurements=on
  G_profile : Lookup_n-D  NumberOfTableDimensions=1  BreakpointsForDimension1=t_day  Table=G_day  ExtrapMethod=Clip  InternalRulePriority=Speed  RndMeth=Simplest
  Gate : DataTypeConversion  OutDataTypeStr=double  SaturateOnIntegerOverflow=off  RndMeth=Floor
  Hour_of_day : Gain  Gain=1/t_hour
  I_meas : spsCurrentMeasurementLib/Current Measurement  PhasorSimulation=off  OutputType=Complex  PSBequivalent=0
  L : spsSeriesRLCBranchLib/Series RLC Branch  LConnTagsString=__new0  RConnTagsString=__new0  BranchType=L  Resistance=1  Inductance=0.30e-3  SetiL0=off  InitialCurrent=0  Capacitance=1e-6  Setx0=off  InitialVoltage=0  Measurements=None
  Mode : Switch  Criteria=u2 ~= 0  SaturateOnIntegerOverflow=off  InputSameDT=off
  NOCT_heating : Gain  Gain=(45-20)/800
  PI_CV : slpidlib/PID Controller  Controller=PI  Form=Parallel  TimeDomain=Discrete-time  UseExternalTs=off  SampleTime=0.0001  IntegratorMethod=Forward Euler  FilterMethod=Forward Euler  ControllerParametersSource=internal  P=0.001  I=0.05  UseKiTs=off  D=0  UseExternalDerivativeSource=off  N=100  UseFilter=on  TunerSelectOption=Transfer Function Based (PID Tuner App)  InitialConditionSource=internal  InitialConditionForIntegrator=0  InitialConditionForFilter=0  DifferentiatorICPrevScaledInput=0  ExternalReset=none  TrackingMode=off  Kt=1  LimitOutput=off  SatLimitsSource=internal  UpperSaturationLimit=inf  LowerSaturationLimit=-inf  LinearizeAsGain=off  AntiWindupMode=none  Kb=1  LimitIntegrator=off  UpperIntegratorSaturationLimit=inf  LowerIntegratorSaturationLimit=-inf  POutMin=[]  POutMax=[]  IOutMin=[]  IOutMax=[]  DOutMin=[]  DOutMax=[]  NOutMin=[]  NOutMax=[]  SumOutMin=[]  SumOutMax=[]  SaturationOutMin=[]  SaturationOutMax=[]  PParamMin=[]  PParamMax=[]  IParamMin=[]  IParamMax=[]  DParamMin=[]  DParamMax=[]  NParamMin=[]  NParamMax=[]  KbParamMin=[]  KbParamMax=[]  KtParamMin=[]  KtParamMax=[]  KbOutMin=[]  KbOutMax=[]  KtOutMin=[]  KtOutMax=[]  IntegratorOutMin=[]  IntegratorOutMax=[]  FilterOutMin=[]  FilterOutMax=[]  SumI1OutMin=[]  SumI1OutMax=[]  SumI2OutMin=[]  SumI2OutMax=[]  SumI3OutMin=[]  SumI3OutMax=[]  SumI4OutMin=[]  SumI4OutMax=[]  SumDOutMin=[]  SumDOutMax=[]  DifferentiatorOutMin=[]  DifferentiatorOutMax=[]  FilterDiffOutCoefMin=[]  FilterDiffOutCoefMax=[]  ReciprocalOutMin=[]  ReciprocalOutMax=[]  SumDenOutMin=[]  SumDenOutMax=[]  SumNumOutMin=[]  SumNumOutMax=[]  DivideOutMin=[]  DivideOutMax=[]  UdiffTsProdOutMin=[]  UdiffTsProdOutMax=[]  NTsProdOutMin=[]  NTsProdOutMax=[]  UintegralTsProdOutMin=[]  UintegralTsProdOutMax=[]  UngainTsProdOutMin=[]  UngainTsProdOutMax=[]  ClampingZeroOutDataTypeStr=Inherit: Inherit via back propagation  ClampingZeroOutMin=[]  ClampingZeroOutMax=[]  FilterDenConstantOutDataTypeStr=Inherit: Inherit via back propagation  FilterDenConstantOutMin=[]  FilterDenConstantOutMax=[]  PCopyOutDataTypeStr=Inherit: Inherit via back propagation  PCopyOutMin=[]  PCopyOutMax=[]  NCopyOutDataTypeStr=Inherit: Inherit via back propagation  NCopyOutMin=[]  NCopyOutMax=[]  IntegratorContinuousStateAttributes=''  IntegratorStateMustResolveToSignalObject=off  IntegratorRTWStateStorageClass=Auto  FilterContinuousStateAttributes=''  FilterStateMustResolveToSignalObject=off  FilterRTWStateStorageClass=Auto  ParallelPVariant=InternalParameters  IdealPVariant=Disabled  IVariant=InternalParameters  DVariant=Disabled  IntegratorVariant=Discrete  SatVariant=Disabled  AWVariant=Passthrough  PCopyVariant=Disabled  TRVariant=Disabled  FdbkBlocksVariant=Forward  IdealPFdbkVariant=Disabled  SatFdbkVariant=Disabled  DerivativeFilterVariant=Disabled  NVariant=Disabled  NCopyVariant=Disabled_SignalSpec  FilterICVariant=Disabled  IntegratorICVariant=InternalICs  ExternalResetVariant=Disabled  TRSumVariant=Passthrough  SumFdbkVariant=Disabled  SumVariant=Sum_PI  TsampFilterVariant=InternalTs  TsampNgainVariant=Passthrough  TsampIntegralVariant=Disabled_SignalSpec  ExternalSaturationOutDataTypeStr=Inherit: Same as second input  DerivativeSourceVariant=Disabled  PreIntVariant=InternalPreInt
      settings: LibrarySourceBlock=simulink/Discrete/Discrete PID Controller
  PV : spsPVArrayLib/PV Array  Npar=8  Nser=6  PlotType=array @ 1000 W/m2 & specified temperatures  S_vec="[ 1000  500  100 ]"  Temp_C_vec="[ 45 25  ]"  ModuleName=User-defined  PlotWhenSelected=off  Pm=400  Ncell=72  Voc=48  Isc=10.5  Vm=40  Im=10  beta_Voc_pc=-0.36099  alpha_Isc_pc=0.102  beta_Voc=-0.17328  alpha_Isc=0.01071  IL=10.576  I0=3.9433e-10  nI=1.0809  Rsh=821.7644  Rs=0.20021  RobustModel=off  RobustCellTemperature=313.3991  BAL=on  Tc=1e-6  Tfilter=5e-5
  PV_Scope : Scope  NumInputPorts=5
      settings: ActiveDisplayYMinimum=-29.860009730532969  ActiveDisplayYMaximum=268.7400875747968  DataLoggingDecimation=100  DataLoggingVariableName=pvdata
  PWM : RelationalOperator  Operator=>  OutDataTypeStr=boolean  RndMeth=Simplest  InputSameDT=off
  P_PV : Product
  PandO : MATLAB Function  TreatAsAtomicUnit=on
  SOC_full : Relay  OnSwitchValue=98  OffSwitchValue=95
  SW : spsIdealSwitchLib/Ideal Switch  Ron=0.001  Lon=0  IC=0  Rs=1e5  Cs=inf  Measurements=on
  Sat_CV : Saturate  UpperLimit=0.85  LowerLimit=0.05
  T_cell : Sum
  Tamb_profile : Lookup_n-D  NumberOfTableDimensions=1  BreakpointsForDimension1=t_day  Table=T_amb_day  ExtrapMethod=Clip  InternalRulePriority=Speed  RndMeth=Simplest
  V_err : Sum  Inputs=+-
  V_meas_PV : spsVoltageMeasurementLib/Voltage Measurement  PhasorSimulation=off  OutputType=Complex  PSBequivalent=0
  V_meas_bus : spsVoltageMeasurementLib/Voltage Measurement  PhasorSimulation=off  OutputType=Complex  PSBequivalent=0
  V_ref : Constant  Value=400
  Weather_15min : ZeroOrderHold  SampleTime=Ts_fc
  Weather_Scope : Scope  NumInputPorts=2
      settings: ActiveDisplayYMinimum=-116.6156432836914  ActiveDisplayYMaximum=1049.5407895532228  DataLoggingVariableName=wxdata
  ZOH_I : ZeroOrderHold  SampleTime=0.0001
  ZOH_V : ZeroOrderHold  SampleTime=0.0001
  DC_Bus+ : PMIOPort  Side=Right
  DC_Bus- : PMIOPort  Port=2  Side=Right
  m1 : Outport
  m2 : Outport  Port=2
  wires:
  V_meas_bus/1 -> V_err/2, PV_Scope/5
  P_PV/1 -> PV_Scope/3
  I_meas/1 -> P_PV/2, PV_Scope/2, ZOH_I/1
  T_cell/1 -> Weather_Scope/2, PV/2
  NOCT_heating/1 -> T_cell/1
  PI_CV/1 -> Sat_CV/1
  Gate/1 -> SW/1
  Hour_of_day/1 -> Weather_15min/1
  V_err/1 -> PI_CV/1
  Carrier/1 -> PWM/2
  ZOH_V/1 -> PandO/1(Vpv)
  PandO/1(D) -> Mode/3
  Clock/1 -> Hour_of_day/1
  V_ref/1 -> V_err/1
  ZOH_I/1 -> PandO/2(Ipv)
  Tamb_profile/1 -> T_cell/2
  Weather_15min/1 -> G_profile/1, Tamb_profile/1
  G_profile/1 -> PV/1, Weather_Scope/1, NOCT_heating/1
  PWM/1 -> Gate/1
  V_meas_PV/1 -> ZOH_V/1, P_PV/1, PV_Scope/1
  Sat_CV/1 -> Mode/1
  Mode/1 -> PWM/1, PV_Scope/4
  SW/1 -> m2/1
  PV/1 -> m1/1
  [SoC_Battery] -> SOC_full/1
  SOC_full/1 -> Mode/2
  connections:
  C_out/LConn1 -- V_meas_bus/LConn1 -- DC_Bus+/RConn1 -- D/RConn1
  C_in/RConn1 -- SW/RConn1 -- C_out/RConn1 -- PV/RConn2 -- V_meas_PV/LConn2 -- V_meas_bus/LConn2 -- DC_Bus-/RConn1
  C_in/LConn1 -- V_meas_PV/LConn1 -- I_meas/RConn1 -- L/LConn1
  SW/LConn1 -- D/LConn1 -- L/RConn1
  PV/RConn1 -- I_meas/LConn1

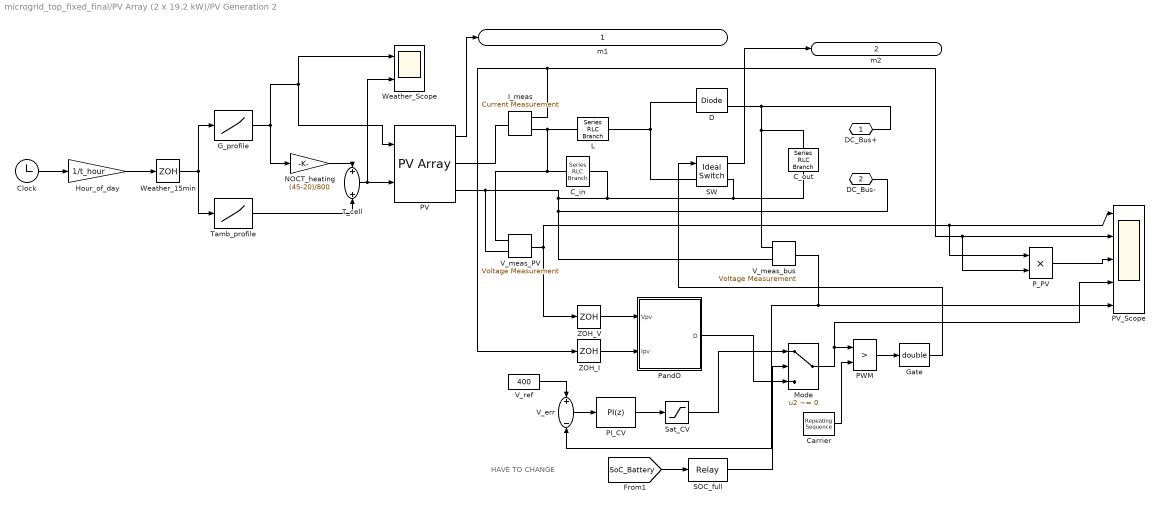
== system microgrid_top_fixed_final/PV Array (2 x 19.2 kW)/PV Generation 2 ==
  note: HAVE TO CHANGE
  C_in : spsSeriesRLCBranchLib/Series RLC Branch  LConnTagsString=__new0  RConnTagsString=__new0  BranchType=C  Resistance=1  Inductance=1e-3  SetiL0=off  InitialCurrent=0  Capacitance=270e-6  Setx0=off  InitialVoltage=0  Measurements=None
  C_out : spsSeriesRLCBranchLib/Series RLC Branch  LConnTagsString=__new0  RConnTagsString=__new0  BranchType=C  Resistance=1  Inductance=1e-3  SetiL0=off  InitialCurrent=0  Capacitance=270e-6  Setx0=off  InitialVoltage=0  Measurements=None
  Carrier : simulink/Sources/Repeating Sequence  rep_seq_t=[0 5e-05]  rep_seq_y=[0 1]
  Clock : Clock
  D : spsDiodeLib/Diode  Ron=0.001  Lon=0  Vf=0.8  IC=0  UseSnubber=0  Rs=500  Cs=250e-9  Measurements=on
  G_profile : Lookup_n-D  NumberOfTableDimensions=1  BreakpointsForDimension1=t_day  Table=G_day  ExtrapMethod=Clip  InternalRulePriority=Speed  RndMeth=Simplest
  Gate : DataTypeConversion  OutDataTypeStr=double  SaturateOnIntegerOverflow=off  RndMeth=Floor
  Hour_of_day : Gain  Gain=1/t_hour
  I_meas : spsCurrentMeasurementLib/Current Measurement  PhasorSimulation=off  OutputType=Complex  PSBequivalent=0
  L : spsSeriesRLCBranchLib/Series RLC Branch  LConnTagsString=__new0  RConnTagsString=__new0  BranchType=L  Resistance=1  Inductance=0.30e-3  SetiL0=off  InitialCurrent=0  Capacitance=1e-6  Setx0=off  InitialVoltage=0  Measurements=None
  Mode : Switch  Criteria=u2 ~= 0  SaturateOnIntegerOverflow=off  InputSameDT=off
  NOCT_heating : Gain  Gain=(45-20)/800
  PI_CV : slpidlib/PID Controller  Controller=PI  Form=Parallel  TimeDomain=Discrete-time  UseExternalTs=off  SampleTime=0.0001  IntegratorMethod=Forward Euler  FilterMethod=Forward Euler  ControllerParametersSource=internal  P=0.001  I=0.05  UseKiTs=off  D=0  UseExternalDerivativeSource=off  N=100  UseFilter=on  TunerSelectOption=Transfer Function Based (PID Tuner App)  InitialConditionSource=internal  InitialConditionForIntegrator=0  InitialConditionForFilter=0  DifferentiatorICPrevScaledInput=0  ExternalReset=none  TrackingMode=off  Kt=1  LimitOutput=off  SatLimitsSource=internal  UpperSaturationLimit=inf  LowerSaturationLimit=-inf  LinearizeAsGain=off  AntiWindupMode=none  Kb=1  LimitIntegrator=off  UpperIntegratorSaturationLimit=inf  LowerIntegratorSaturationLimit=-inf  POutMin=[]  POutMax=[]  IOutMin=[]  IOutMax=[]  DOutMin=[]  DOutMax=[]  NOutMin=[]  NOutMax=[]  SumOutMin=[]  SumOutMax=[]  SaturationOutMin=[]  SaturationOutMax=[]  PParamMin=[]  PParamMax=[]  IParamMin=[]  IParamMax=[]  DParamMin=[]  DParamMax=[]  NParamMin=[]  NParamMax=[]  KbParamMin=[]  KbParamMax=[]  KtParamMin=[]  KtParamMax=[]  KbOutMin=[]  KbOutMax=[]  KtOutMin=[]  KtOutMax=[]  IntegratorOutMin=[]  IntegratorOutMax=[]  FilterOutMin=[]  FilterOutMax=[]  SumI1OutMin=[]  SumI1OutMax=[]  SumI2OutMin=[]  SumI2OutMax=[]  SumI3OutMin=[]  SumI3OutMax=[]  SumI4OutMin=[]  SumI4OutMax=[]  SumDOutMin=[]  SumDOutMax=[]  DifferentiatorOutMin=[]  DifferentiatorOutMax=[]  FilterDiffOutCoefMin=[]  FilterDiffOutCoefMax=[]  ReciprocalOutMin=[]  ReciprocalOutMax=[]  SumDenOutMin=[]  SumDenOutMax=[]  SumNumOutMin=[]  SumNumOutMax=[]  DivideOutMin=[]  DivideOutMax=[]  UdiffTsProdOutMin=[]  UdiffTsProdOutMax=[]  NTsProdOutMin=[]  NTsProdOutMax=[]  UintegralTsProdOutMin=[]  UintegralTsProdOutMax=[]  UngainTsProdOutMin=[]  UngainTsProdOutMax=[]  ClampingZeroOutDataTypeStr=Inherit: Inherit via back propagation  ClampingZeroOutMin=[]  ClampingZeroOutMax=[]  FilterDenConstantOutDataTypeStr=Inherit: Inherit via back propagation  FilterDenConstantOutMin=[]  FilterDenConstantOutMax=[]  PCopyOutDataTypeStr=Inherit: Inherit via back propagation  PCopyOutMin=[]  PCopyOutMax=[]  NCopyOutDataTypeStr=Inherit: Inherit via back propagation  NCopyOutMin=[]  NCopyOutMax=[]  IntegratorContinuousStateAttributes=''  IntegratorStateMustResolveToSignalObject=off  IntegratorRTWStateStorageClass=Auto  FilterContinuousStateAttributes=''  FilterStateMustResolveToSignalObject=off  FilterRTWStateStorageClass=Auto  ParallelPVariant=InternalParameters  IdealPVariant=Disabled  IVariant=InternalParameters  DVariant=Disabled  IntegratorVariant=Discrete  SatVariant=Disabled  AWVariant=Passthrough  PCopyVariant=Disabled  TRVariant=Disabled  FdbkBlocksVariant=Forward  IdealPFdbkVariant=Disabled  SatFdbkVariant=Disabled  DerivativeFilterVariant=Disabled  NVariant=Disabled  NCopyVariant=Disabled_SignalSpec  FilterICVariant=Disabled  IntegratorICVariant=InternalICs  ExternalResetVariant=Disabled  TRSumVariant=Passthrough  SumFdbkVariant=Disabled  SumVariant=Sum_PI  TsampFilterVariant=InternalTs  TsampNgainVariant=Passthrough  TsampIntegralVariant=Disabled_SignalSpec  ExternalSaturationOutDataTypeStr=Inherit: Same as second input  DerivativeSourceVariant=Disabled  PreIntVariant=InternalPreInt
      settings: LibrarySourceBlock=simulink/Discrete/Discrete PID Controller
  PV : spsPVArrayLib/PV Array  Npar=8  Nser=6  PlotType=array @ 1000 W/m2 & specified temperatures  S_vec="[ 1000  500  100 ]"  Temp_C_vec="[ 45 25  ]"  ModuleName=User-defined  PlotWhenSelected=off  Pm=400  Ncell=72  Voc=48  Isc=10.5  Vm=40  Im=10  beta_Voc_pc=-0.36099  alpha_Isc_pc=0.102  beta_Voc=-0.17328  alpha_Isc=0.01071  IL=10.576  I0=3.9433e-10  nI=1.0809  Rsh=821.7644  Rs=0.20021  RobustModel=off  RobustCellTemperature=313.3991  BAL=on  Tc=1e-6  Tfilter=5e-5
  PV_Scope : Scope  NumInputPorts=5
      settings: ActiveDisplayYMinimum=-29.860009730532969  ActiveDisplayYMaximum=268.7400875747968  DataLoggingDecimation=100  DataLoggingVariableName=pvdata
  PWM : RelationalOperator  Operator=>  OutDataTypeStr=boolean  RndMeth=Simplest  InputSameDT=off
  P_PV : Product
  PandO : MATLAB Function  TreatAsAtomicUnit=on
  SOC_full : Relay  OnSwitchValue=98  OffSwitchValue=95
  SW : spsIdealSwitchLib/Ideal Switch  Ron=0.001  Lon=0  IC=0  Rs=1e5  Cs=inf  Measurements=on
  Sat_CV : Saturate  UpperLimit=0.85  LowerLimit=0.05
  T_cell : Sum
  Tamb_profile : Lookup_n-D  NumberOfTableDimensions=1  BreakpointsForDimension1=t_day  Table=T_amb_day  ExtrapMethod=Clip  InternalRulePriority=Speed  RndMeth=Simplest
  V_err : Sum  Inputs=+-
  V_meas_PV : spsVoltageMeasurementLib/Voltage Measurement  PhasorSimulation=off  OutputType=Complex  PSBequivalent=0
  V_meas_bus : spsVoltageMeasurementLib/Voltage Measurement  PhasorSimulation=off  OutputType=Complex  PSBequivalent=0
  V_ref : Constant  Value=400
  Weather_15min : ZeroOrderHold  SampleTime=Ts_fc
  Weather_Scope : Scope  NumInputPorts=2
      settings: ActiveDisplayYMinimum=-116.6156432836914  ActiveDisplayYMaximum=1049.5407895532228  DataLoggingVariableName=wxdata
  ZOH_I : ZeroOrderHold  SampleTime=0.0001
  ZOH_V : ZeroOrderHold  SampleTime=0.0001
  DC_Bus+ : PMIOPort  Side=Right
  DC_Bus- : PMIOPort  Port=2  Side=Right
  m1 : Outport
  m2 : Outport  Port=2
  wires:
  PV/1 -> m1/1
  SW/1 -> m2/1
  Mode/1 -> PV_Scope/4, PWM/1
  Sat_CV/1 -> Mode/1
  V_meas_PV/1 -> PV_Scope/1, P_PV/1, ZOH_V/1
  PWM/1 -> Gate/1
  G_profile/1 -> NOCT_heating/1, Weather_Scope/1, PV/1
  Weather_15min/1 -> Tamb_profile/1, G_profile/1
  Tamb_profile/1 -> T_cell/2
  ZOH_I/1 -> PandO/2(Ipv)
  V_ref/1 -> V_err/1
  Clock/1 -> Hour_of_day/1
  PandO/1(D) -> Mode/3
  ZOH_V/1 -> PandO/1(Vpv)
  Carrier/1 -> PWM/2
  V_err/1 -> PI_CV/1
  Hour_of_day/1 -> Weather_15min/1
  Gate/1 -> SW/1
  PI_CV/1 -> Sat_CV/1
  NOCT_heating/1 -> T_cell/1
  T_cell/1 -> PV/2, Weather_Scope/2
  I_meas/1 -> ZOH_I/1, PV_Scope/2, P_PV/2
  P_PV/1 -> PV_Scope/3
  V_meas_bus/1 -> PV_Scope/5, V_err/2
  [SoC_Battery] -> SOC_full/1
  SOC_full/1 -> Mode/2
  connections:
  PV/RConn1 -- I_meas/LConn1
  L/RConn1 -- D/LConn1 -- SW/LConn1
  L/LConn1 -- I_meas/RConn1 -- V_meas_PV/LConn1 -- C_in/LConn1
  DC_Bus-/RConn1 -- V_meas_bus/LConn2 -- V_meas_PV/LConn2 -- PV/RConn2 -- C_out/RConn1 -- SW/RConn1 -- C_in/RConn1
  D/RConn1 -- DC_Bus+/RConn1 -- V_meas_bus/LConn1 -- C_out/LConn1

== system microgrid_top_fixed_final/Supercapacitor + DC-DC/Bidirectional DC-DC converter For Supercapacitor ==
  D_Q1 : Inport
  D_Q2 : Inport  Port=2
  L_Bidirectional : spsSeriesRLCBranchLib/Series RLC Branch  LConnTagsString=__new0  RConnTagsString=__new0  BranchType=RL  Resistance=0.05  Inductance=0.355e-3  SetiL0=off  InitialCurrent=0  Capacitance=1e-6  Setx0=off  InitialVoltage=0  Measurements=None
  Q1 : spsIGBTDiodeLib/IGBT//Diode  Ron=1e-3  Rs=1e5  Cs=inf  Measurements=on
  Q2 : spsIGBTDiodeLib/IGBT//Diode  Ron=1e-3  Rs=1e5  Cs=inf  Measurements=on
  Terminator : Terminator
  Terminator1 : Terminator
  High + : PMIOPort  Side=Left
  Low + : PMIOPort  Port=2  Side=Right
  High - : PMIOPort  Port=3  Side=Right
  Low - : PMIOPort  Port=4  Side=Right
  wires:
  D_Q2/1 -> Q2/1
  D_Q1/1 -> Q1/1
  Q1/1 -> Terminator/1
  Q2/1 -> Terminator1/1
  connections:
  High -/RConn1 -- Low -/RConn1 -- Q2/RConn1
  Low +/RConn1 -- L_Bidirectional/RConn1
  Q2/LConn1 -- L_Bidirectional/LConn1 -- Q1/RConn1
  High +/RConn1 -- Q1/LConn1
